simulink model "course_lab6_lead1"  (R2024b)
settings: Solver=ode45  StartTime=0.0  StopTime=5  MaxStep=0.003333333333333334  RelTol=1e-7  AbsTol=1e-9
model workspace (MAT data in the model file):
  A = 1
  K = 10
  Kv = 20
  alpha = 2.46730897709
  den = [0.08160435262 1.16320870524 10.0537260716 40]
  frequency = 1
  num = [0 0 8.05372607156 40]
  plant_den = [1 2 0]
  plant_num = [0 0 40]
  reserve = 8
  targetPM = 35
  web_input = timeseries
  web_input.Name = 'unnamed'
  web_input.DataInfo = tsdata.datametadata
  web_input.DataInfo.Interpolation = tsdata.interpolation
  web_input.DataInfo.Interpolation.Fhandle : function handle (value not decoded)
  web_input.DataInfo.Interpolation.Name = 'linear'
  web_input.TimeInfo = tsdata.timemetadata
  web_input.TimeInfo.Length = 1501
  web_input.TimeInfo.DuplicateTimes = 0
  web_input.TimeInfo.Time_ = [0 0.00333333333333 0.00666666666667 0.01 0.0133333333333 0.0166666666667 0.02 0.0233333333333 0.0266666666667 0.03 0.0333333333333 0.0366666666667 ... (1501 elements, 1501x1)]
  web_input.TimeInfo.Initialized = 1
  web_input.QualityInfo = tsdata.qualmetadata
  web_input.Data_ = [1 1 1 1 1 1 1 1 1 1 1 1 ... (1501 elements, 1501x1)]
  wp = 12.2542483078
  wz = 4.96664520802
settings Model: Creator=33657  LastModifiedBy=33657

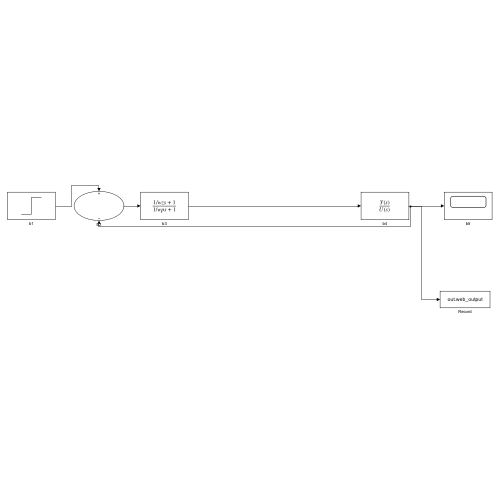
[thumbnail: Simulink's stored preview of the top-level diagram]
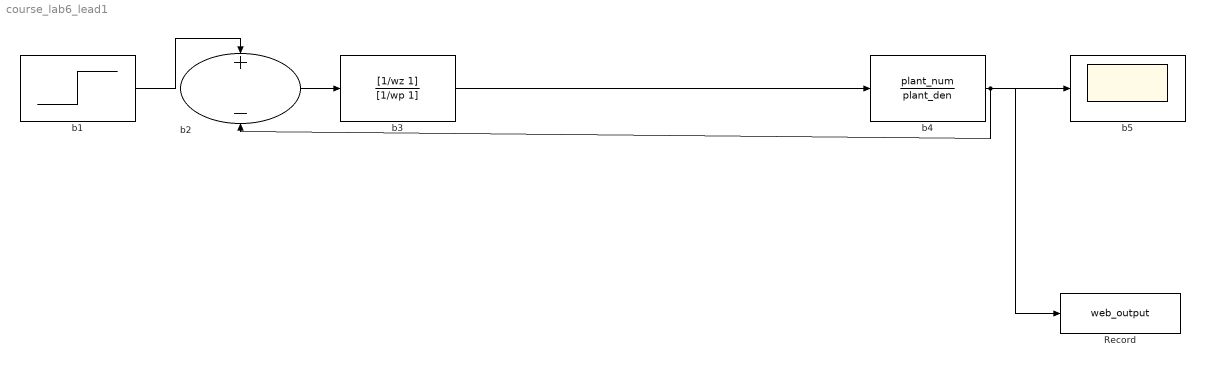
== system course_lab6_lead1 ==
  Record : ToWorkspace  VariableName=web_output  SaveFormat=Timeseries  SampleTime=-1
  b1 : Step  Time=0  After=A  SampleTime=0
  b2 : Sum  Inputs=+-
  b3 : TransferFcn  Numerator=[1/wz 1]  Denominator=[1/wp 1]
  b4 : TransferFcn  Numerator=plant_num  Denominator=plant_den
  b5 : Scope
  wires:
  b1/1 -> b2/1
  b2/1 -> b3/1
  b3/1 -> b4/1
  b4/1 -> b2/2, b5/1, Record/1
